simulink model "Comb8_final_chain"  (R2022b)
settings: Solver=VariableStepDiscrete  StartTime=0.0  StopTime=0.01  RelTol=1e-3
libraries: dspsigops x24, dspsrcs4 x2, simulink x1
settings Model: Creator=ASAA  LastModifiedBy=ASAA
settings DataIOCC: ReturnWorkspaceOutputs=off
settings DebuggingCC: SignalRangeChecking=warning  ParameterOverflowMsg=none

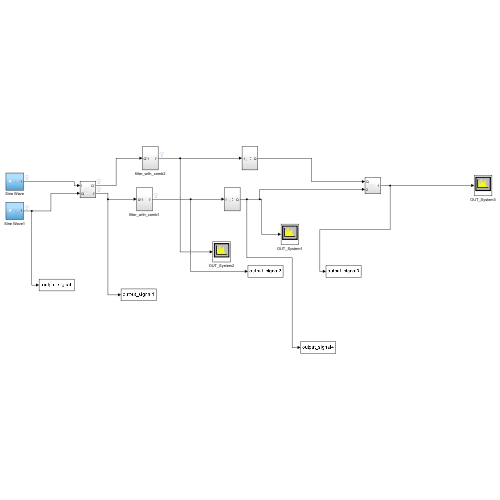
[thumbnail: Simulink's stored preview of the top-level diagram]
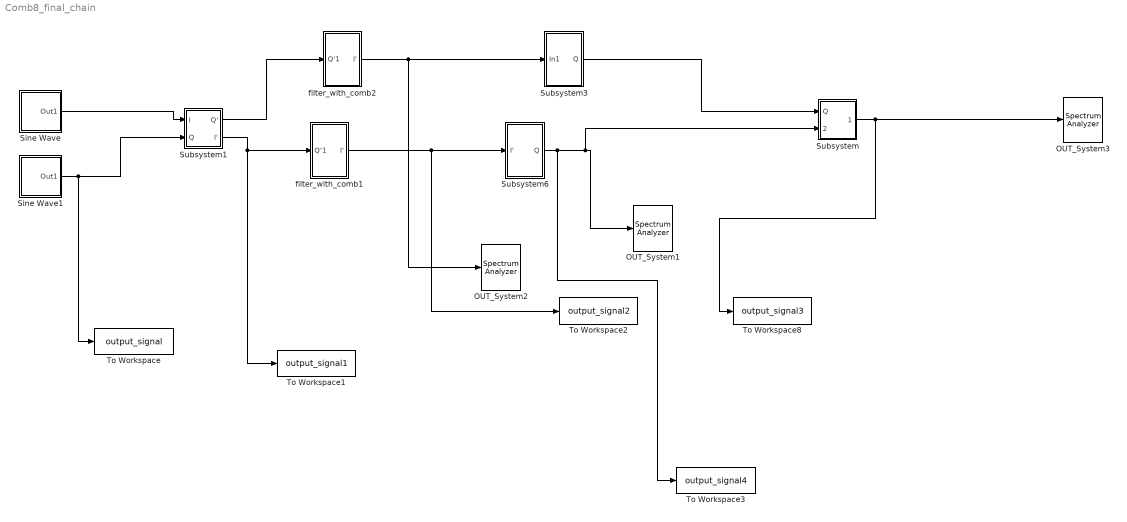
== system Comb8_final_chain ==
  OUT_System1 : SpectrumAnalyzer
  OUT_System2 : SpectrumAnalyzer
  OUT_System3 : SpectrumAnalyzer
  Sine Wave : Subsystem  Tag=DecoupledSystem
  Sine Wave1 : Subsystem  Tag=DecoupledSystem
  Subsystem : Subsystem
  Subsystem1 : Subsystem
  Subsystem3 : Subsystem
  Subsystem6 : Subsystem
  To Workspace : ToWorkspace  VariableName=output_signal  SaveFormat=Timeseries  SampleTime=-1
  To Workspace1 : ToWorkspace  VariableName=output_signal1  SaveFormat=Timeseries  SampleTime=-1
  To Workspace2 : ToWorkspace  VariableName=output_signal2  SaveFormat=Timeseries  SampleTime=-1
  To Workspace3 : ToWorkspace  VariableName=output_signal4  SaveFormat=Timeseries  SampleTime=-1
  To Workspace8 : ToWorkspace  VariableName=output_signal3  SaveFormat=Timeseries  SampleTime=-1
  filter_with_comb1 : Subsystem
  filter_with_comb2 : Subsystem
  wires:
  Sine Wave1/1(Out1) -> Subsystem1/2(Q), To Workspace/1
  Sine Wave/1(Out1) -> Subsystem1/1(I)
  Subsystem6/1(Q) -> Subsystem/2(In2), OUT_System1/1, To Workspace3/1
  Subsystem1/2(I') -> filter_with_comb1/1(Q'1), To Workspace1/1
  filter_with_comb2/1(I') -> OUT_System2/1, Subsystem3/1(In1)
  Subsystem1/1(Q') -> filter_with_comb2/1(Q'1)
  filter_with_comb1/1(I') -> To Workspace2/1, Subsystem6/1(I')
  Subsystem/1(Out1) -> To Workspace8/1, OUT_System3/1
  Subsystem3/1(Q) -> Subsystem/1(Q)

== system Comb8_final_chain/Sine Wave ==
  ReplicaOfSource : dspsrcs4/Sine Wave  Amplitude=0.631  Frequency=100e3  Phase=0  SampleMode=Discrete  OutComplex=Real  CompMethod=Trigonometric fcn  TableSize=Speed  SampleTime=1/3.125e6  SamplesPerFrame=1  ResetState=Restart at time zero  OutputFrames=off  dataType=double  wordLen=16  udDataType=sfix(16)  fracBitsMode=Best precision  numFracBits=15  OutDataTypeStr=double  LastOutDataTypeStr=double
  Out1 : Outport  LockScale=on
  wires:
  ReplicaOfSource/1 -> Out1/1

== system Comb8_final_chain/Sine Wave1 ==
  ReplicaOfSource : dspsrcs4/Sine Wave  Amplitude=0.631  Frequency=100e3  Phase=pi/2  SampleMode=Discrete  OutComplex=Real  CompMethod=Trigonometric fcn  TableSize=Speed  SampleTime=1/3.125e6  SamplesPerFrame=1  ResetState=Restart at time zero  OutputFrames=off  dataType=double  wordLen=16  udDataType=sfix(16)  fracBitsMode=Best precision  numFracBits=15  OutDataTypeStr=double  LastOutDataTypeStr=double
  Out1 : Outport  LockScale=on
  wires:
  ReplicaOfSource/1 -> Out1/1

== system Comb8_final_chain/Subsystem ==
  Q : Inport
  In2 : Inport  Port=2
  -I(t) : Gain  Gain=-1
  -Q(t) : Gain  Gain=-1
  Counter : simulink/Sources/Counter Limited  uplimit=3  tsamp=1/400e6
  Multiport Switch (MUX) : MultiPortSwitch  DataPortOrder=Zero-based contiguous  Inputs=4  zeroidx=on  SaturateOnIntegerOverflow=off  InputSameDT=off
  Out1 : Outport
  wires:
  Q/1 -> Multiport Switch (MUX)/2, -I(t)/1
  Counter/1 -> Multiport Switch (MUX)/1
  -Q(t)/1 -> Multiport Switch (MUX)/3
  In2/1 -> Multiport Switch (MUX)/5, -Q(t)/1
  -I(t)/1 -> Multiport Switch (MUX)/4
  Multiport Switch (MUX)/1 -> Out1/1

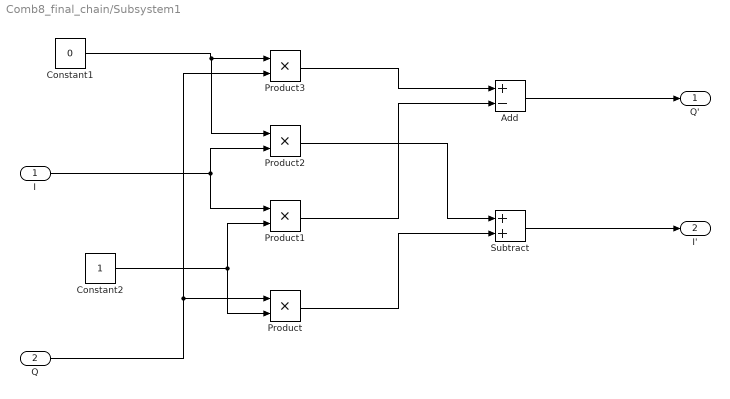
== system Comb8_final_chain/Subsystem1 ==
  I : Inport
  Q : Inport  Port=2
  Add : Sum  Inputs=+-
  Constant1 : Constant  Value=0
  Constant2 : Constant
  Product{,1..3} (4 alike) : Product
  Subtract : Sum
  Q' : Outport
  I' : Outport  Port=2
  wires:
  Constant2/1 -> Product/2, Product1/2
  Add/1 -> Q'/1
  Constant1/1 -> Product2/1, Product3/1
  Product3/1 -> Add/1
  Product2/1 -> Subtract/1
  Product1/1 -> Add/2
  Product/1 -> Subtract/2
  Subtract/1 -> I'/1
  I/1 -> Product1/1, Product2/2
  Q/1 -> Product3/2, Product/1

== system Comb8_final_chain/Subsystem3 ==
  In1 : Inport
  Gain : Gain  Gain=2  SaturateOnIntegerOverflow=on
  Sign : Signum
  Sum : Sum  Inputs=|+-  RndMeth=Nearest  SaturateOnIntegerOverflow=on
  Sum1 : Sum  Inputs=|++-  SaturateOnIntegerOverflow=on
  Unit Delay : UnitDelay  SampleTime=1e-8  HasFrameUpgradeWarning=on
  Unit Delay1 : UnitDelay  SampleTime=1e-8  HasFrameUpgradeWarning=on
  Q : Outport
  wires:
  Sign/1 -> Q/1, Sum/2
  Sum1/1 -> Sign/1, Sum/1
  Sum/1 -> Unit Delay1/1
  Unit Delay1/1 -> Unit Delay/1, Gain/1
  Gain/1 -> Sum1/2
  In1/1 -> Sum1/1
  Unit Delay/1 -> Sum1/3

== system Comb8_final_chain/Subsystem6 ==
  I' : Inport
  Gain : Gain  Gain=2
  Sign : Signum
  Sum : Sum  Inputs=|+-
  Sum1 : Sum  Inputs=|++-
  Unit Delay : UnitDelay  SampleTime=1e-8  HasFrameUpgradeWarning=on
  Unit Delay1 : UnitDelay  SampleTime=1e-8  HasFrameUpgradeWarning=on
  Q : Outport
  wires:
  Sign/1 -> Q/1, Sum/2
  Sum1/1 -> Sign/1, Sum/1
  Sum/1 -> Unit Delay1/1
  Unit Delay1/1 -> Unit Delay/1, Gain/1
  Gain/1 -> Sum1/2
  I'/1 -> Sum1/1
  Unit Delay/1 -> Sum1/3

== system Comb8_final_chain/filter_with_comb1 ==
  Q'1 : Inport
  Gain : Gain  Gain=1/512
  Stage_1 : Subsystem
  stage_3 : Subsystem
  stage_4 : Subsystem
  I' : Outport
  wires:
  stage_4/1(Out1) -> stage_3/1(In1)
  Q'1/1 -> stage_4/1(Q')
  stage_3/1(Q') -> Stage_1/1(In1)
  Stage_1/1(I') -> Gain/1
  Gain/1 -> I'/1

== system Comb8_final_chain/filter_with_comb2 ==
  Q'1 : Inport
  Gain : Gain  Gain=1/512
  Stage_1 : Subsystem
  stage_3 : Subsystem
  stage_4 : Subsystem
  I' : Outport
  wires:
  stage_4/1(Out1) -> stage_3/1(In1)
  Q'1/1 -> stage_4/1(Q')
  stage_3/1(Q') -> Stage_1/1(In1)
  Stage_1/1(I') -> Gain/1
  Gain/1 -> I'/1

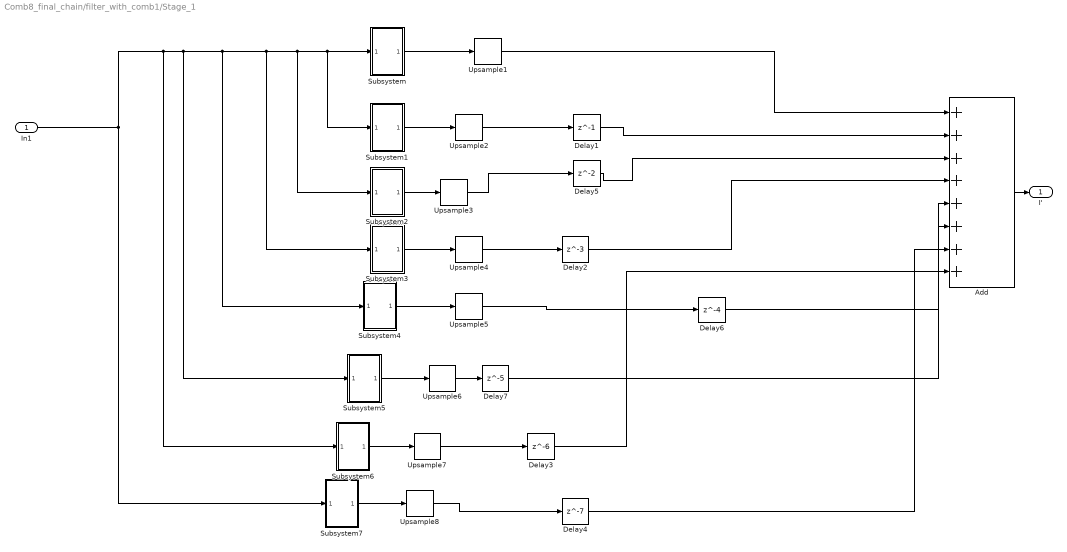
== system Comb8_final_chain/filter_with_comb1/Stage_1 ==
  In1 : Inport
  Add : Sum  Inputs=++++++++
  Delay1 : Delay  DelayLength=1  InitialCondition=0
  Delay2 : Delay  DelayLength=3  InitialCondition=0
  Delay3 : Delay  DelayLength=6  InitialCondition=0
  Delay4 : Delay  DelayLength=7  InitialCondition=0
  Delay5 : Delay  InitialCondition=0
  Delay6 : Delay  DelayLength=4  InitialCondition=0
  Delay7 : Delay  DelayLength=5  InitialCondition=0
  Subsystem : Subsystem
  Subsystem1 : Subsystem
  Subsystem2 : Subsystem
  Subsystem3 : Subsystem
  Subsystem4 : Subsystem
  Subsystem5 : Subsystem
  Subsystem6 : Subsystem
  Subsystem7 : Subsystem
  Upsample{1..8} (8 alike) : dspsigops/Upsample  N=8  phase=0  RateOptions=Allow multirate processing  ic=0  mode=Unused parameter value
  I' : Outport
  wires:
  In1/1 -> Subsystem6/1(In2), Subsystem5/1(In2), Subsystem4/1(In2), Subsystem3/1(In2), Subsystem2/1(In2), Subsystem1/1(In2), Subsystem/1(In1), Subsystem7/1(In2)
  Subsystem/1(Out1) -> Upsample1/1
  Add/1 -> I'/1
  Delay1/1 -> Add/2
  Delay5/1 -> Add/3
  Delay2/1 -> Add/4
  Delay6/1 -> Add/5
  Delay7/1 -> Add/6
  Delay3/1 -> Add/8
  Delay4/1 -> Add/7
  Subsystem5/1(Out2) -> Upsample6/1
  Subsystem4/1(Out2) -> Upsample5/1
  Subsystem3/1(Out2) -> Upsample4/1
  Subsystem2/1(Out2) -> Upsample3/1
  Subsystem1/1(Out2) -> Upsample2/1
  Subsystem7/1(Out2) -> Upsample8/1
  Subsystem6/1(Out2) -> Upsample7/1
  Upsample1/1 -> Add/1
  Upsample2/1 -> Delay1/1
  Upsample3/1 -> Delay5/1
  Upsample4/1 -> Delay2/1
  Upsample5/1 -> Delay6/1
  Upsample6/1 -> Delay7/1
  Upsample7/1 -> Delay3/1
  Upsample8/1 -> Delay4/1

== system Comb8_final_chain/filter_with_comb1/stage_3 ==
  In1 : Inport
  Add1 : Sum
  Delay1 : Delay  DelayLength=1  InitialCondition=0
  Delay3 : Delay  DelayLength=9  InitialCondition=0
  Gain1 : Gain  Gain=0.5000
  Subsystem : Subsystem
  Upsample2 : dspsigops/Upsample  N=2  phase=0  RateOptions=Allow multirate processing  ic=0  mode=Unused parameter value
  Upsample3 : dspsigops/Upsample  N=2  phase=0  RateOptions=Allow multirate processing  ic=0  mode=Unused parameter value
  Q' : Outport
  wires:
  Gain1/1 -> Upsample2/1
  Add1/1 -> Q'/1
  Delay3/1 -> Gain1/1
  Subsystem/1(Out1) -> Upsample3/1
  Upsample2/1 -> Delay1/1
  In1/1 -> Delay3/1, Subsystem/1(In1)
  Upsample3/1 -> Add1/1
  Delay1/1 -> Add1/2

== system Comb8_final_chain/filter_with_comb1/stage_4 ==
  Q' : Inport
  Add : Sum
  Delay1 : Delay  DelayLength=15  InitialCondition=0
  Delay2 : Delay  DelayLength=1  InitialCondition=0
  Gain : Gain  Gain=0.5000
  Subsystem1 : Subsystem
  Upsample : dspsigops/Upsample  N=2  phase=0  RateOptions=Allow multirate processing  ic=0  mode=Unused parameter value
  Upsample1 : dspsigops/Upsample  N=2  phase=0  RateOptions=Allow multirate processing  ic=0  mode=Unused parameter value
  Out1 : Outport
  wires:
  Add/1 -> Out1/1
  Gain/1 -> Upsample1/1
  Delay1/1 -> Gain/1
  Subsystem1/1(Out2) -> Upsample/1
  Q'/1 -> Subsystem1/1(Q'), Delay1/1
  Upsample1/1 -> Delay2/1
  Upsample/1 -> Add/1
  Delay2/1 -> Add/2

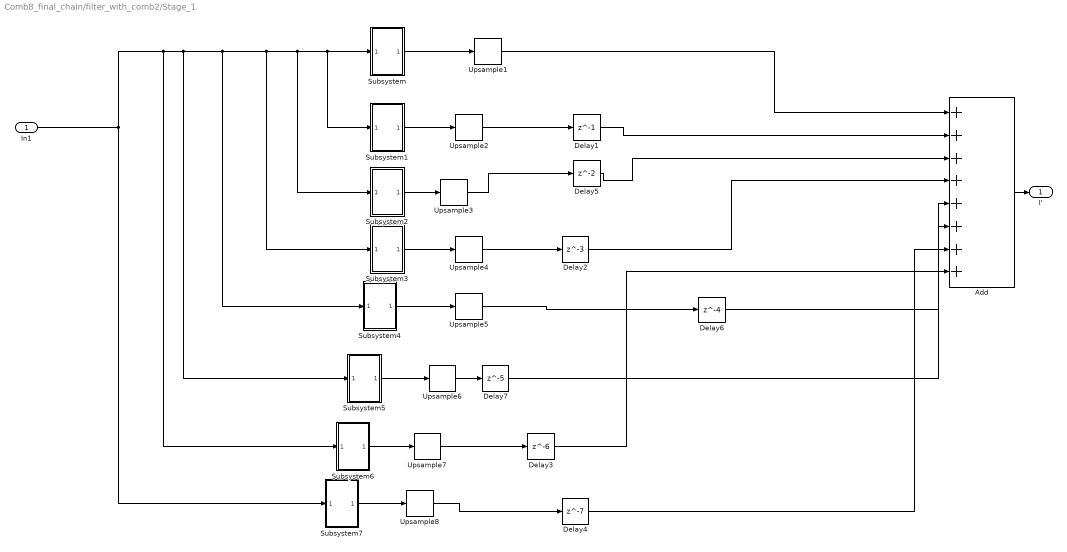
== system Comb8_final_chain/filter_with_comb2/Stage_1 ==
  In1 : Inport
  Add : Sum  Inputs=++++++++
  Delay1 : Delay  DelayLength=1  InitialCondition=0
  Delay2 : Delay  DelayLength=3  InitialCondition=0
  Delay3 : Delay  DelayLength=6  InitialCondition=0
  Delay4 : Delay  DelayLength=7  InitialCondition=0
  Delay5 : Delay  InitialCondition=0
  Delay6 : Delay  DelayLength=4  InitialCondition=0
  Delay7 : Delay  DelayLength=5  InitialCondition=0
  Subsystem : Subsystem
  Subsystem1 : Subsystem
  Subsystem2 : Subsystem
  Subsystem3 : Subsystem
  Subsystem4 : Subsystem
  Subsystem5 : Subsystem
  Subsystem6 : Subsystem
  Subsystem7 : Subsystem
  Upsample{1..8} (8 alike) : dspsigops/Upsample  N=8  phase=0  RateOptions=Allow multirate processing  ic=0  mode=Unused parameter value
  I' : Outport
  wires:
  In1/1 -> Subsystem6/1(In2), Subsystem5/1(In2), Subsystem4/1(In2), Subsystem3/1(In2), Subsystem2/1(In2), Subsystem1/1(In2), Subsystem/1(In1), Subsystem7/1(In2)
  Subsystem/1(Out1) -> Upsample1/1
  Add/1 -> I'/1
  Delay1/1 -> Add/2
  Delay5/1 -> Add/3
  Delay2/1 -> Add/4
  Delay6/1 -> Add/5
  Delay7/1 -> Add/6
  Delay3/1 -> Add/8
  Delay4/1 -> Add/7
  Subsystem5/1(Out2) -> Upsample6/1
  Subsystem4/1(Out2) -> Upsample5/1
  Subsystem3/1(Out2) -> Upsample4/1
  Subsystem2/1(Out2) -> Upsample3/1
  Subsystem1/1(Out2) -> Upsample2/1
  Subsystem7/1(Out2) -> Upsample8/1
  Subsystem6/1(Out2) -> Upsample7/1
  Upsample1/1 -> Add/1
  Upsample2/1 -> Delay1/1
  Upsample3/1 -> Delay5/1
  Upsample4/1 -> Delay2/1
  Upsample5/1 -> Delay6/1
  Upsample6/1 -> Delay7/1
  Upsample7/1 -> Delay3/1
  Upsample8/1 -> Delay4/1

== system Comb8_final_chain/filter_with_comb2/stage_3 ==
  In1 : Inport
  Add1 : Sum
  Delay1 : Delay  DelayLength=1  InitialCondition=0
  Delay3 : Delay  DelayLength=9  InitialCondition=0
  Gain1 : Gain  Gain=0.5000
  Subsystem : Subsystem
  Upsample2 : dspsigops/Upsample  N=2  phase=0  RateOptions=Allow multirate processing  ic=0  mode=Unused parameter value
  Upsample3 : dspsigops/Upsample  N=2  phase=0  RateOptions=Allow multirate processing  ic=0  mode=Unused parameter value
  Q' : Outport
  wires:
  Gain1/1 -> Upsample2/1
  Add1/1 -> Q'/1
  Delay3/1 -> Gain1/1
  Subsystem/1(Out1) -> Upsample3/1
  Upsample2/1 -> Delay1/1
  In1/1 -> Delay3/1, Subsystem/1(In1)
  Upsample3/1 -> Add1/1
  Delay1/1 -> Add1/2

== system Comb8_final_chain/filter_with_comb2/stage_4 ==
  Q' : Inport
  Add : Sum
  Delay1 : Delay  DelayLength=15  InitialCondition=0
  Delay2 : Delay  DelayLength=1  InitialCondition=0
  Gain : Gain  Gain=0.5000
  Subsystem1 : Subsystem
  Upsample : dspsigops/Upsample  N=2  phase=0  RateOptions=Allow multirate processing  ic=0  mode=Unused parameter value
  Upsample1 : dspsigops/Upsample  N=2  phase=0  RateOptions=Allow multirate processing  ic=0  mode=Unused parameter value
  Out1 : Outport
  wires:
  Add/1 -> Out1/1
  Gain/1 -> Upsample1/1
  Delay1/1 -> Gain/1
  Subsystem1/1(Out2) -> Upsample/1
  Q'/1 -> Subsystem1/1(Q'), Delay1/1
  Upsample1/1 -> Delay2/1
  Upsample/1 -> Add/1
  Delay2/1 -> Add/2

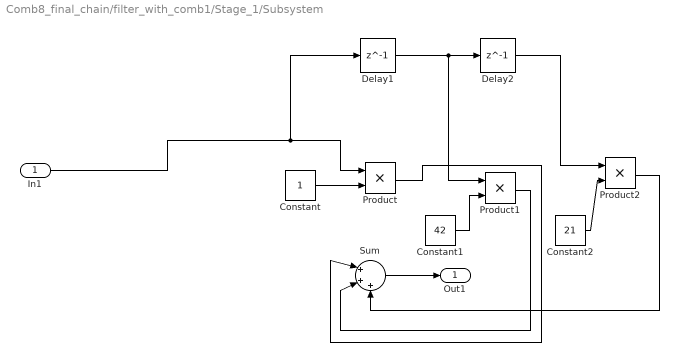
== system Comb8_final_chain/filter_with_comb1/Stage_1/Subsystem ==
  In1 : Inport
  Constant : Constant
  Constant1 : Constant  Value=42
  Constant2 : Constant  Value=21
  Delay1 : Delay  DelayLength=1  InitialCondition=0
  Delay2 : Delay  DelayLength=1  InitialCondition=0
  Product : Product
  Product1 : Product
  Product2 : Product
  Sum : Sum  Inputs=|+++
  Out1 : Outport
  wires:
  Constant1/1 -> Product1/2
  In1/1 -> Product/1, Delay1/1
  Product1/1 -> Sum/2
  Product/1 -> Sum/1
  Sum/1 -> Out1/1
  Constant/1 -> Product/2
  Delay1/1 -> Delay2/1, Product1/1
  Delay2/1 -> Product2/1
  Constant2/1 -> Product2/2
  Product2/1 -> Sum/3

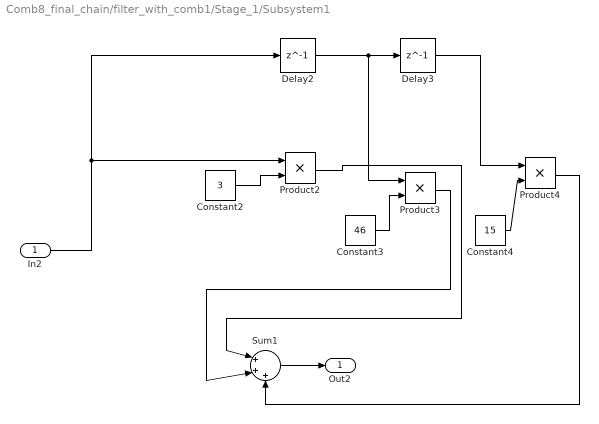
== system Comb8_final_chain/filter_with_comb1/Stage_1/Subsystem1 ==
  In2 : Inport
  Constant2 : Constant  Value=3
  Constant3 : Constant  Value=46
  Constant4 : Constant  Value=15
  Delay2 : Delay  DelayLength=1  InitialCondition=0
  Delay3 : Delay  DelayLength=1  InitialCondition=0
  Product2 : Product
  Product3 : Product
  Product4 : Product
  Sum1 : Sum  Inputs=|+++
  Out2 : Outport
  wires:
  Delay3/1 -> Product4/1
  Delay2/1 -> Delay3/1, Product3/1
  Sum1/1 -> Out2/1
  Constant2/1 -> Product2/2
  Product2/1 -> Sum1/1
  Constant3/1 -> Product3/2
  Product3/1 -> Sum1/2
  Constant4/1 -> Product4/2
  In2/1 -> Delay2/1, Product2/1
  Product4/1 -> Sum1/3

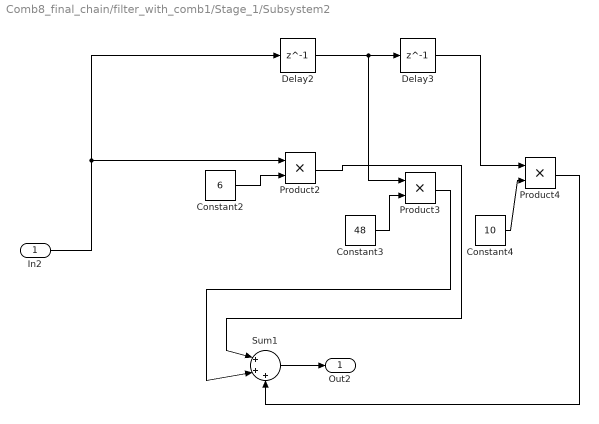
== system Comb8_final_chain/filter_with_comb1/Stage_1/Subsystem2 ==
  In2 : Inport
  Constant2 : Constant  Value=6
  Constant3 : Constant  Value=48
  Constant4 : Constant  Value=10
  Delay2 : Delay  DelayLength=1  InitialCondition=0
  Delay3 : Delay  DelayLength=1  InitialCondition=0
  Product2 : Product
  Product3 : Product
  Product4 : Product
  Sum1 : Sum  Inputs=|+++
  Out2 : Outport
  wires:
  In2/1 -> Delay2/1, Product2/1
  Constant4/1 -> Product4/2
  Product2/1 -> Sum1/1
  Constant3/1 -> Product3/2
  Constant2/1 -> Product2/2
  Delay2/1 -> Delay3/1, Product3/1
  Product3/1 -> Sum1/2
  Sum1/1 -> Out2/1
  Delay3/1 -> Product4/1
  Product4/1 -> Sum1/3

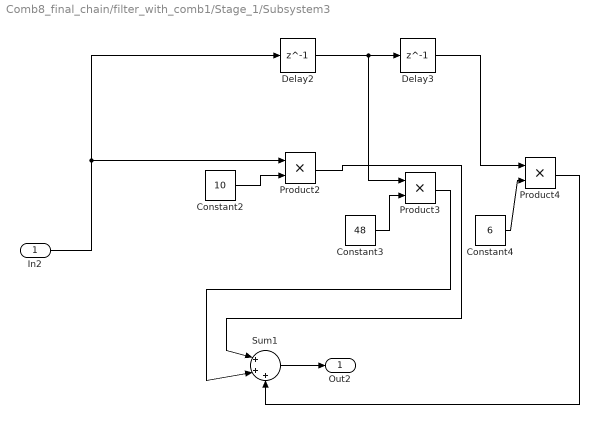
== system Comb8_final_chain/filter_with_comb1/Stage_1/Subsystem3 ==
  In2 : Inport
  Constant2 : Constant  Value=10
  Constant3 : Constant  Value=48
  Constant4 : Constant  Value=6
  Delay2 : Delay  DelayLength=1  InitialCondition=0
  Delay3 : Delay  DelayLength=1  InitialCondition=0
  Product2 : Product
  Product3 : Product
  Product4 : Product
  Sum1 : Sum  Inputs=|+++
  Out2 : Outport
  wires:
  In2/1 -> Delay2/1, Product2/1
  Constant4/1 -> Product4/2
  Product2/1 -> Sum1/1
  Constant3/1 -> Product3/2
  Constant2/1 -> Product2/2
  Delay2/1 -> Delay3/1, Product3/1
  Product3/1 -> Sum1/2
  Sum1/1 -> Out2/1
  Delay3/1 -> Product4/1
  Product4/1 -> Sum1/3

== system Comb8_final_chain/filter_with_comb1/Stage_1/Subsystem4 ==
  In2 : Inport
  Constant2 : Constant  Value=15
  Constant3 : Constant  Value=46
  Constant4 : Constant  Value=3
  Delay2 : Delay  DelayLength=1  InitialCondition=0
  Delay3 : Delay  DelayLength=1  InitialCondition=0
  Product2 : Product
  Product3 : Product
  Product4 : Product
  Sum1 : Sum  Inputs=|+++++
  Out2 : Outport
  wires:
  In2/1 -> Delay2/1, Product2/1
  Product4/1 -> Sum1/4
  Constant4/1 -> Product4/2
  Product2/1 -> Sum1/1
  Constant3/1 -> Product3/2
  Constant2/1 -> Product2/2
  Delay2/1 -> Delay3/1, Product3/1
  Product3/1 -> Sum1/2
  Sum1/1 -> Out2/1
  Delay3/1 -> Product4/1

== system Comb8_final_chain/filter_with_comb1/Stage_1/Subsystem5 ==
  In2 : Inport
  Constant2 : Constant  Value=21
  Constant3 : Constant  Value=42
  Constant4 : Constant
  Delay2 : Delay  DelayLength=1  InitialCondition=0
  Delay3 : Delay  DelayLength=1  InitialCondition=0
  Product2 : Product
  Product3 : Product
  Product4 : Product
  Sum1 : Sum  Inputs=|+++
  Out2 : Outport
  wires:
  In2/1 -> Delay2/1, Product2/1
  Constant4/1 -> Product4/2
  Product2/1 -> Sum1/1
  Constant3/1 -> Product3/2
  Constant2/1 -> Product2/2
  Delay2/1 -> Delay3/1, Product3/1
  Product3/1 -> Sum1/2
  Sum1/1 -> Out2/1
  Delay3/1 -> Product4/1
  Product4/1 -> Sum1/3

== system Comb8_final_chain/filter_with_comb1/Stage_1/Subsystem6 ==
  In2 : Inport
  Constant2 : Constant  Value=28
  Constant3 : Constant  Value=36
  Delay2 : Delay  DelayLength=1  InitialCondition=0
  Product2 : Product
  Product3 : Product
  Sum1 : Sum  Inputs=|++
  Out2 : Outport
  wires:
  In2/1 -> Delay2/1, Product2/1
  Product2/1 -> Sum1/1
  Constant3/1 -> Product3/2
  Constant2/1 -> Product2/2
  Delay2/1 -> Product3/1
  Product3/1 -> Sum1/2
  Sum1/1 -> Out2/1

== system Comb8_final_chain/filter_with_comb1/Stage_1/Subsystem7 ==
  In2 : Inport
  Constant2 : Constant  Value=36
  Constant3 : Constant  Value=28
  Delay2 : Delay  DelayLength=1  InitialCondition=0
  Product2 : Product
  Product3 : Product
  Sum1 : Sum  Inputs=|++
  Out2 : Outport
  wires:
  In2/1 -> Delay2/1, Product2/1
  Product2/1 -> Sum1/1
  Constant3/1 -> Product3/2
  Constant2/1 -> Product2/2
  Delay2/1 -> Product3/1
  Product3/1 -> Sum1/2
  Sum1/1 -> Out2/1

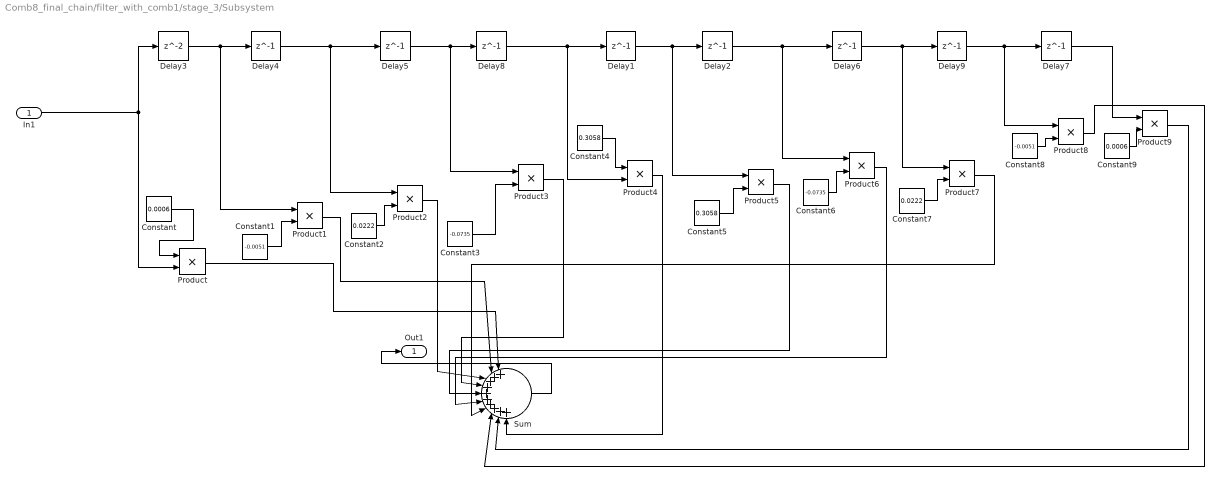
== system Comb8_final_chain/filter_with_comb1/stage_3/Subsystem ==
  In1 : Inport
  Constant : Constant  Value=0.0006
  Constant1 : Constant  Value=-0.0051
  Constant2 : Constant  Value=0.0222
  Constant3 : Constant  Value=-0.0735
  Constant4 : Constant  Value=0.3058
  Constant5 : Constant  Value=0.3058
  Constant6 : Constant  Value=-0.0735
  Constant7 : Constant  Value=0.0222
  Constant8 : Constant  Value=-0.0051
  Constant9 : Constant  Value=0.0006
  Delay{1..2,4..9} (8 alike) : Delay  DelayLength=1  InitialCondition=0
  Delay3 : Delay  InitialCondition=0
  Product{,1..9} (10 alike) : Product
  Sum : Sum  Inputs=|++++++++++
  Out1 : Outport
  wires:
  Product/1 -> Sum/1
  Product2/1 -> Sum/3
  Delay3/1 -> Product1/1, Delay4/1
  Sum/1 -> Out1/1
  Delay4/1 -> Product2/1, Delay5/1
  Product3/1 -> Sum/4
  In1/1 -> Product/2, Delay3/1
  Constant2/1 -> Product2/2
  Constant3/1 -> Product3/2
  Constant/1 -> Product/1
  Product1/1 -> Sum/2
  Constant1/1 -> Product1/2
  Delay5/1 -> Delay8/1, Product3/1
  Constant7/1 -> Product7/2
  Constant5/1 -> Product5/2
  Constant4/1 -> Product4/1
  Delay6/1 -> Product7/1, Delay9/1
  Delay2/1 -> Delay6/1, Product6/1
  Delay1/1 -> Delay2/1, Product5/1
  Constant6/1 -> Product6/2
  Constant8/1 -> Product8/2
  Constant9/1 -> Product9/2
  Delay7/1 -> Product9/1
  Product5/1 -> Sum/5
  Product6/1 -> Sum/6
  Product7/1 -> Sum/7
  Product8/1 -> Sum/8
  Product9/1 -> Sum/9
  Product4/1 -> Sum/10
  Delay8/1 -> Product4/2, Delay1/1
  Delay9/1 -> Product8/1, Delay7/1

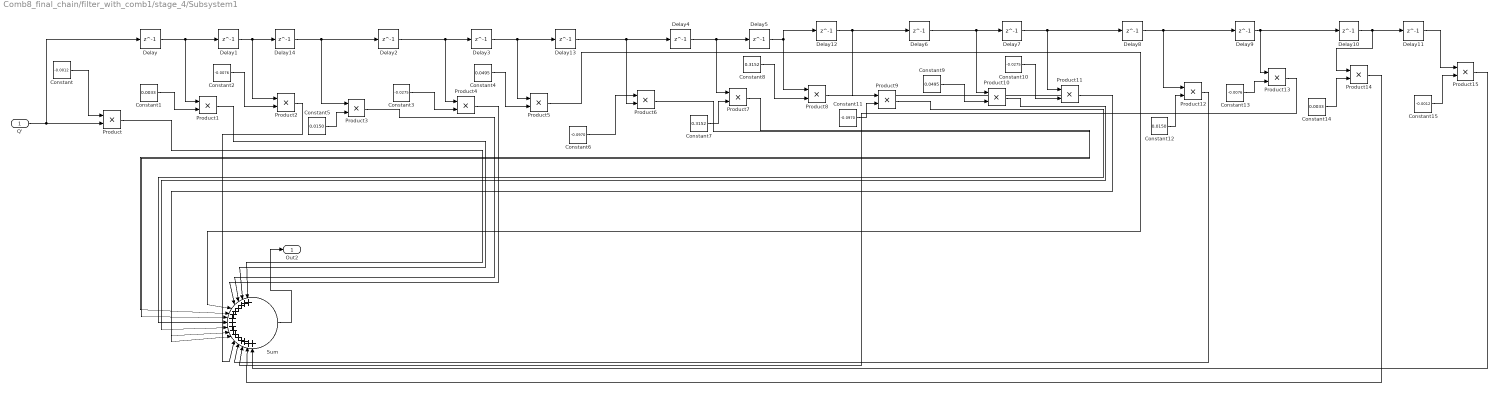
== system Comb8_final_chain/filter_with_comb1/stage_4/Subsystem1 ==
  Q' : Inport
  Constant : Constant  Value=-0.0012
  Constant1 : Constant  Value=0.0033
  Constant10 : Constant  Value=-0.0275
  Constant11 : Constant  Value=-0.0970
  Constant12 : Constant  Value=0.0150
  Constant13 : Constant  Value=-0.0076
  Constant14 : Constant  Value=0.0033
  Constant15 : Constant  Value=-0.0012
  Constant2 : Constant  Value=-0.0076
  Constant3 : Constant  Value=-0.0275
  Constant4 : Constant  Value=0.0495
  Constant5 : Constant  Value=0.0150
  Constant6 : Constant  Value=-0.0970
  Constant7 : Constant  Value=0.3152
  Constant8 : Constant  Value=0.3152
  Constant9 : Constant  Value=0.0495
  Delay{,1..14} (15 alike) : Delay  DelayLength=1  InitialCondition=0
  Product{,1..15} (16 alike) : Product
  Sum : Sum  Inputs=|++++++++++++++++
  Out2 : Outport
  wires:
  Constant1/1 -> Product1/2
  Delay2/1 -> Delay3/1, Product4/1
  Constant10/1 -> Product11/2
  Constant9/1 -> Product10/2
  Delay/1 -> Delay1/1, Product1/1
  Delay4/1 -> Delay5/1, Product7/1
  Constant3/1 -> Product4/2
  Product8/1 -> Sum/11
  Product6/1 -> Sum/6
  Delay1/1 -> Product2/1, Delay14/1
  Delay5/1 -> Delay12/1, Product8/1
  Constant8/1 -> Product8/2
  Q'/1 -> Delay/1, Product/2
  Delay6/1 -> Delay7/1, Product10/1
  Constant/1 -> Product/1
  Constant11/1 -> Product9/2
  Product10/1 -> Sum/9
  Delay7/1 -> Delay8/1, Product11/1
  Product9/1 -> Sum/8
  Delay3/1 -> Product5/1, Delay13/1
  Constant4/1 -> Product5/2
  Product3/1 -> Sum/3
  Product5/1 -> Sum/5
  Constant2/1 -> Product2/2
  Constant5/1 -> Product3/2
  Constant7/1 -> Product7/2
  Product11/1 -> Sum/10
  Constant6/1 -> Product6/1
  Product/1 -> Sum/1
  Product1/1 -> Sum/2
  Product7/1 -> Sum/7
  Product4/1 -> Sum/4
  Sum/1 -> Out2/1
  Product2/1 -> Sum/12
  Constant12/1 -> Product12/2
  Delay8/1 -> Product12/1, Delay9/1
  Constant13/1 -> Product13/2
  Delay9/1 -> Delay10/1, Product13/1
  Constant14/1 -> Product14/2
  Delay10/1 -> Delay11/1, Product14/1
  Delay11/1 -> Product15/1
  Constant15/1 -> Product15/2
  Product12/1 -> Sum/13
  Product13/1 -> Sum/14
  Product14/1 -> Sum/15
  Product15/1 -> Sum/16
  Delay12/1 -> Delay6/1, Product9/1
  Delay13/1 -> Delay4/1, Product6/2
  Delay14/1 -> Delay2/1, Product3/1

== system Comb8_final_chain/filter_with_comb2/Stage_1/Subsystem ==
  In1 : Inport
  Constant : Constant
  Constant1 : Constant  Value=42
  Constant2 : Constant  Value=21
  Delay1 : Delay  DelayLength=1  InitialCondition=0
  Delay2 : Delay  DelayLength=1  InitialCondition=0
  Product : Product
  Product1 : Product
  Product2 : Product
  Sum : Sum  Inputs=|+++
  Out1 : Outport
  wires:
  Constant1/1 -> Product1/2
  In1/1 -> Product/1, Delay1/1
  Product1/1 -> Sum/2
  Product/1 -> Sum/1
  Sum/1 -> Out1/1
  Constant/1 -> Product/2
  Delay1/1 -> Delay2/1, Product1/1
  Delay2/1 -> Product2/1
  Constant2/1 -> Product2/2
  Product2/1 -> Sum/3

== system Comb8_final_chain/filter_with_comb2/Stage_1/Subsystem1 ==
  In2 : Inport
  Constant2 : Constant  Value=3
  Constant3 : Constant  Value=46
  Constant4 : Constant  Value=15
  Delay2 : Delay  DelayLength=1  InitialCondition=0
  Delay3 : Delay  DelayLength=1  InitialCondition=0
  Product2 : Product
  Product3 : Product
  Product4 : Product
  Sum1 : Sum  Inputs=|+++
  Out2 : Outport
  wires:
  Delay3/1 -> Product4/1
  Delay2/1 -> Delay3/1, Product3/1
  Sum1/1 -> Out2/1
  Constant2/1 -> Product2/2
  Product2/1 -> Sum1/1
  Constant3/1 -> Product3/2
  Product3/1 -> Sum1/2
  Constant4/1 -> Product4/2
  In2/1 -> Delay2/1, Product2/1
  Product4/1 -> Sum1/3

== system Comb8_final_chain/filter_with_comb2/Stage_1/Subsystem2 ==
  In2 : Inport
  Constant2 : Constant  Value=6
  Constant3 : Constant  Value=48
  Constant4 : Constant  Value=10
  Delay2 : Delay  DelayLength=1  InitialCondition=0
  Delay3 : Delay  DelayLength=1  InitialCondition=0
  Product2 : Product
  Product3 : Product
  Product4 : Product
  Sum1 : Sum  Inputs=|+++
  Out2 : Outport
  wires:
  In2/1 -> Delay2/1, Product2/1
  Constant4/1 -> Product4/2
  Product2/1 -> Sum1/1
  Constant3/1 -> Product3/2
  Constant2/1 -> Product2/2
  Delay2/1 -> Delay3/1, Product3/1
  Product3/1 -> Sum1/2
  Sum1/1 -> Out2/1
  Delay3/1 -> Product4/1
  Product4/1 -> Sum1/3

== system Comb8_final_chain/filter_with_comb2/Stage_1/Subsystem3 ==
  In2 : Inport
  Constant2 : Constant  Value=10
  Constant3 : Constant  Value=48
  Constant4 : Constant  Value=6
  Delay2 : Delay  DelayLength=1  InitialCondition=0
  Delay3 : Delay  DelayLength=1  InitialCondition=0
  Product2 : Product
  Product3 : Product
  Product4 : Product
  Sum1 : Sum  Inputs=|+++
  Out2 : Outport
  wires:
  In2/1 -> Delay2/1, Product2/1
  Constant4/1 -> Product4/2
  Product2/1 -> Sum1/1
  Constant3/1 -> Product3/2
  Constant2/1 -> Product2/2
  Delay2/1 -> Delay3/1, Product3/1
  Product3/1 -> Sum1/2
  Sum1/1 -> Out2/1
  Delay3/1 -> Product4/1
  Product4/1 -> Sum1/3

== system Comb8_final_chain/filter_with_comb2/Stage_1/Subsystem4 ==
  In2 : Inport
  Constant2 : Constant  Value=15
  Constant3 : Constant  Value=46
  Constant4 : Constant  Value=3
  Delay2 : Delay  DelayLength=1  InitialCondition=0
  Delay3 : Delay  DelayLength=1  InitialCondition=0
  Product2 : Product
  Product3 : Product
  Product4 : Product
  Sum1 : Sum  Inputs=|+++++
  Out2 : Outport
  wires:
  In2/1 -> Delay2/1, Product2/1
  Product4/1 -> Sum1/4
  Constant4/1 -> Product4/2
  Product2/1 -> Sum1/1
  Constant3/1 -> Product3/2
  Constant2/1 -> Product2/2
  Delay2/1 -> Delay3/1, Product3/1
  Product3/1 -> Sum1/2
  Sum1/1 -> Out2/1
  Delay3/1 -> Product4/1

== system Comb8_final_chain/filter_with_comb2/Stage_1/Subsystem5 ==
  In2 : Inport
  Constant2 : Constant  Value=21
  Constant3 : Constant  Value=42
  Constant4 : Constant
  Delay2 : Delay  DelayLength=1  InitialCondition=0
  Delay3 : Delay  DelayLength=1  InitialCondition=0
  Product2 : Product
  Product3 : Product
  Product4 : Product
  Sum1 : Sum  Inputs=|+++
  Out2 : Outport
  wires:
  In2/1 -> Delay2/1, Product2/1
  Constant4/1 -> Product4/2
  Product2/1 -> Sum1/1
  Constant3/1 -> Product3/2
  Constant2/1 -> Product2/2
  Delay2/1 -> Delay3/1, Product3/1
  Product3/1 -> Sum1/2
  Sum1/1 -> Out2/1
  Delay3/1 -> Product4/1
  Product4/1 -> Sum1/3

== system Comb8_final_chain/filter_with_comb2/Stage_1/Subsystem6 ==
  In2 : Inport
  Constant2 : Constant  Value=28
  Constant3 : Constant  Value=36
  Delay2 : Delay  DelayLength=1  InitialCondition=0
  Product2 : Product
  Product3 : Product
  Sum1 : Sum  Inputs=|++
  Out2 : Outport
  wires:
  In2/1 -> Delay2/1, Product2/1
  Product2/1 -> Sum1/1
  Constant3/1 -> Product3/2
  Constant2/1 -> Product2/2
  Delay2/1 -> Product3/1
  Product3/1 -> Sum1/2
  Sum1/1 -> Out2/1

== system Comb8_final_chain/filter_with_comb2/Stage_1/Subsystem7 ==
  In2 : Inport
  Constant2 : Constant  Value=36
  Constant3 : Constant  Value=28
  Delay2 : Delay  DelayLength=1  InitialCondition=0
  Product2 : Product
  Product3 : Product
  Sum1 : Sum  Inputs=|++
  Out2 : Outport
  wires:
  In2/1 -> Delay2/1, Product2/1
  Product2/1 -> Sum1/1
  Constant3/1 -> Product3/2
  Constant2/1 -> Product2/2
  Delay2/1 -> Product3/1
  Product3/1 -> Sum1/2
  Sum1/1 -> Out2/1

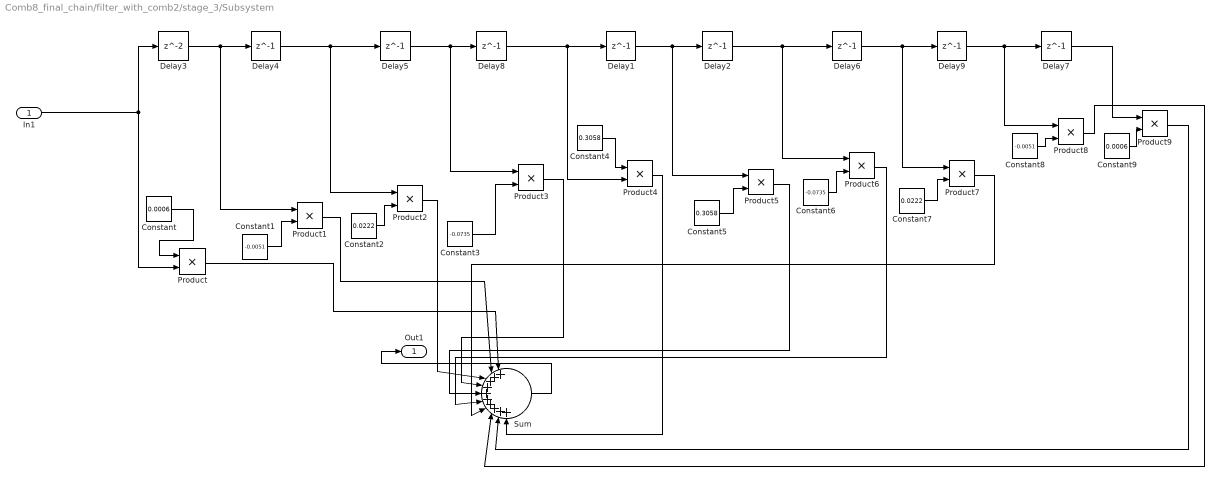
== system Comb8_final_chain/filter_with_comb2/stage_3/Subsystem ==
  In1 : Inport
  Constant : Constant  Value=0.0006
  Constant1 : Constant  Value=-0.0051
  Constant2 : Constant  Value=0.0222
  Constant3 : Constant  Value=-0.0735
  Constant4 : Constant  Value=0.3058
  Constant5 : Constant  Value=0.3058
  Constant6 : Constant  Value=-0.0735
  Constant7 : Constant  Value=0.0222
  Constant8 : Constant  Value=-0.0051
  Constant9 : Constant  Value=0.0006
  Delay{1..2,4..9} (8 alike) : Delay  DelayLength=1  InitialCondition=0
  Delay3 : Delay  InitialCondition=0
  Product{,1..9} (10 alike) : Product
  Sum : Sum  Inputs=|++++++++++
  Out1 : Outport
  wires:
  Product/1 -> Sum/1
  Product2/1 -> Sum/3
  Delay3/1 -> Product1/1, Delay4/1
  Sum/1 -> Out1/1
  Delay4/1 -> Product2/1, Delay5/1
  Product3/1 -> Sum/4
  In1/1 -> Product/2, Delay3/1
  Constant2/1 -> Product2/2
  Constant3/1 -> Product3/2
  Constant/1 -> Product/1
  Product1/1 -> Sum/2
  Constant1/1 -> Product1/2
  Delay5/1 -> Delay8/1, Product3/1
  Constant7/1 -> Product7/2
  Constant5/1 -> Product5/2
  Constant4/1 -> Product4/1
  Delay6/1 -> Product7/1, Delay9/1
  Delay2/1 -> Delay6/1, Product6/1
  Delay1/1 -> Delay2/1, Product5/1
  Constant6/1 -> Product6/2
  Constant8/1 -> Product8/2
  Constant9/1 -> Product9/2
  Delay7/1 -> Product9/1
  Product5/1 -> Sum/5
  Product6/1 -> Sum/6
  Product7/1 -> Sum/7
  Product8/1 -> Sum/8
  Product9/1 -> Sum/9
  Product4/1 -> Sum/10
  Delay8/1 -> Product4/2, Delay1/1
  Delay9/1 -> Product8/1, Delay7/1

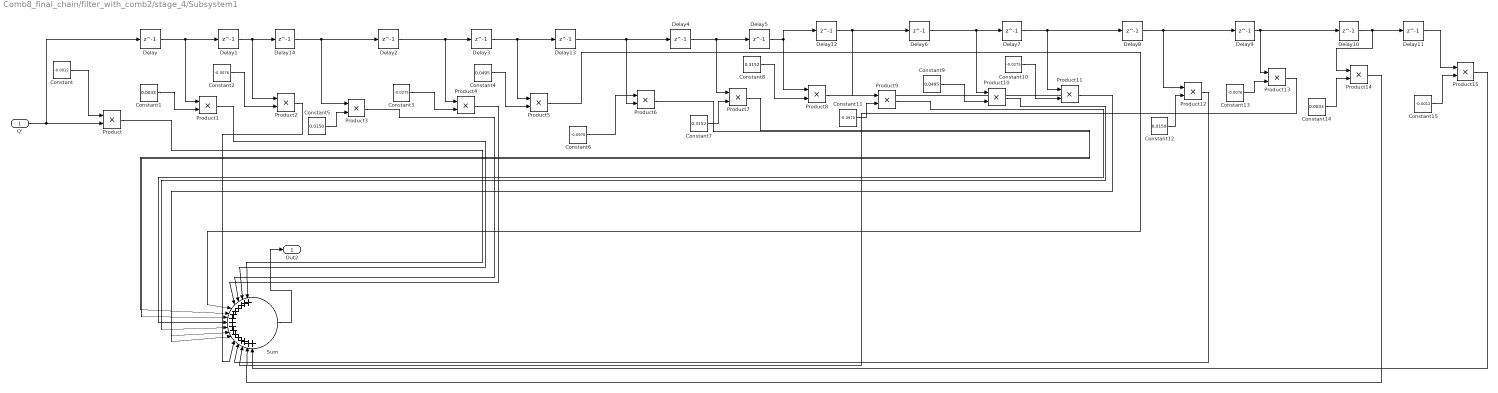
== system Comb8_final_chain/filter_with_comb2/stage_4/Subsystem1 ==
  Q' : Inport
  Constant : Constant  Value=-0.0012
  Constant1 : Constant  Value=0.0033
  Constant10 : Constant  Value=-0.0275
  Constant11 : Constant  Value=-0.0970
  Constant12 : Constant  Value=0.0150
  Constant13 : Constant  Value=-0.0076
  Constant14 : Constant  Value=0.0033
  Constant15 : Constant  Value=-0.0012
  Constant2 : Constant  Value=-0.0076
  Constant3 : Constant  Value=-0.0275
  Constant4 : Constant  Value=0.0495
  Constant5 : Constant  Value=0.0150
  Constant6 : Constant  Value=-0.0970
  Constant7 : Constant  Value=0.3152
  Constant8 : Constant  Value=0.3152
  Constant9 : Constant  Value=0.0495
  Delay{,1..14} (15 alike) : Delay  DelayLength=1  InitialCondition=0
  Product{,1..15} (16 alike) : Product
  Sum : Sum  Inputs=|++++++++++++++++
  Out2 : Outport
  wires:
  Constant1/1 -> Product1/2
  Delay2/1 -> Delay3/1, Product4/1
  Constant10/1 -> Product11/2
  Constant9/1 -> Product10/2
  Delay/1 -> Delay1/1, Product1/1
  Delay4/1 -> Delay5/1, Product7/1
  Constant3/1 -> Product4/2
  Product8/1 -> Sum/11
  Product6/1 -> Sum/6
  Delay1/1 -> Product2/1, Delay14/1
  Delay5/1 -> Delay12/1, Product8/1
  Constant8/1 -> Product8/2
  Q'/1 -> Delay/1, Product/2
  Delay6/1 -> Delay7/1, Product10/1
  Constant/1 -> Product/1
  Constant11/1 -> Product9/2
  Product10/1 -> Sum/9
  Delay7/1 -> Delay8/1, Product11/1
  Product9/1 -> Sum/8
  Delay3/1 -> Product5/1, Delay13/1
  Constant4/1 -> Product5/2
  Product3/1 -> Sum/3
  Product5/1 -> Sum/5
  Constant2/1 -> Product2/2
  Constant5/1 -> Product3/2
  Constant7/1 -> Product7/2
  Product11/1 -> Sum/10
  Constant6/1 -> Product6/1
  Product/1 -> Sum/1
  Product1/1 -> Sum/2
  Product7/1 -> Sum/7
  Product4/1 -> Sum/4
  Sum/1 -> Out2/1
  Product2/1 -> Sum/12
  Constant12/1 -> Product12/2
  Delay8/1 -> Product12/1, Delay9/1
  Constant13/1 -> Product13/2
  Delay9/1 -> Delay10/1, Product13/1
  Constant14/1 -> Product14/2
  Delay10/1 -> Delay11/1, Product14/1
  Delay11/1 -> Product15/1
  Constant15/1 -> Product15/2
  Product12/1 -> Sum/13
  Product13/1 -> Sum/14
  Product14/1 -> Sum/15
  Product15/1 -> Sum/16
  Delay12/1 -> Delay6/1, Product9/1
  Delay13/1 -> Delay4/1, Product6/2
  Delay14/1 -> Delay2/1, Product3/1
